simulink library "cvt_components_lib"  (R2025a)
settings: Solver=VariableStepAuto  StartTime=0.0  StopTime=10.0  RelTol=1e-3
undefined symbols (not defined in the file): HMPST
libraries: fl_lib x15, sdl_lib x5, nesl_utility x2, simulink_extras x1
Description:
  | Copyright 2023-2025 The MathWorks, Inc.
settings Model: Creator=smiller  LastModifiedBy=smiller
settings RTWCC: GPUComputeCapability=3.5

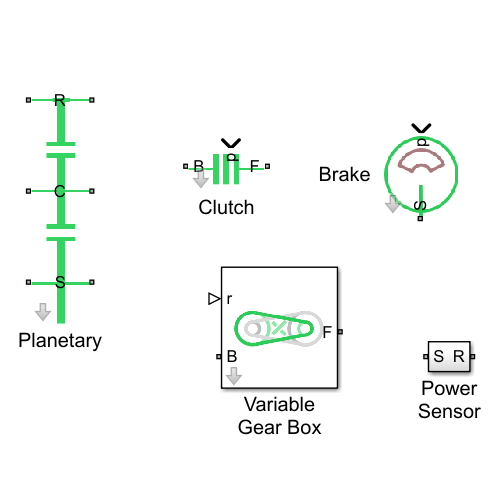
[thumbnail: Simulink's stored preview of the top-level diagram]
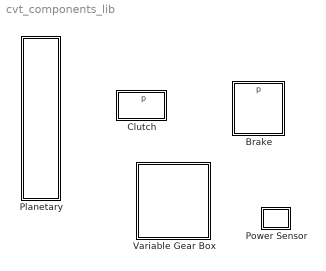
== system cvt_components_lib ==
  Brake : Subsystem  mask(Disk Brake){bore=HMPST.Brake.cylBore, brkwy_vel=HMPST.Brake.vBrk, mu_static=HMPST.Brake.muSta, mu_coulomb=HMPST.Brake.muKin, n_pads=HMPST.Brake.numPads, r_mean=HMPST.Brake.rPad, visc_coef=HMPST.Brake.dVisc, logic2pressure=HMPST.Brake.logic2Press, ts_filt=HMPST.Brake.tsFilt}
      mask prompts: bore "Cylinder bore"; brkwy_vel "Breakaway friction velocity"; mu_static "Static friction coefficient"; mu_coulomb "Coulomb friction coefficient"; n_pads "Number of brake pads"; r_mean "Mean pad radius"; visc_coef "Viscous friction coefficient"; logic2pressure "Logic to Pressure (Pa)"; ts_filt "Filter time constant (sec)"
      mask help: Models a disk brake. Brake actuation dynamics are modeled abstractly as a transfer function.
      mask TypeOptions bore: Brake/bore
      mask TypeOptions brkwy_vel: Brake/brkwy_vel
      mask TypeOptions mu_static: Brake/mu_static
      mask TypeOptions mu_coulomb: Brake/mu_coulomb
      mask TypeOptions n_pads: Brake/n_pads
      mask TypeOptions r_mean: Brake/r_mean
      mask TypeOptions visc_coef: Brake/visc_coef
      mask TypeOptions logic2pressure: Logic to Pressure/Gain
      mask Display: image('sm_wheel_loader_brake1D_IMAGE.png')
  Clutch : Subsystem  mask(Clutch){r_eff=200, nS=8, piston_area=0.0083, mu_static=0.6, mu_coulomb=0.4, w_tol=0.001, pressure_min=100, logic_to_pr_gain=10^6, ts_filt=0.05}
      mask prompts: r_eff "Effective torque radius (mm)"; nS "Number of friction surfaces"; piston_area "Engagement piston area (m^2)"; mu_static "Static friction coefficient (0-1)"; mu_coulomb "Kinetic friction coefficient (0-1)"; w_tol "Clutch velocity tolerance (rad/s)"; pressure_min "Engagement threshold pressure (Pa)"; logic_to_pr_gain "Logic to pressure gain (Pa)"; ts_filt "Filter time constant (sec)"
      mask help: Models a disk clutch. Clutch dynamics for engaging are modeled abstractly as a transfer function.
      settings: PortSchema="{\"entries\":[{\"content\":{\"sides\":[{\"content\":{\"connectorIds\":[\"LConn1\"]},\"type\":\"ConnectorPlacement.EquallySpacedRectSide\",\"uuid\":\"287225fd-8891-4f7c-8f3e-4b5002d781cc\"},{\"content\":{\"connectorIds\":[\"RConn1\"],\"side\":\"RIGHT\"},\"type\":\"ConnectorPlacement.EquallySpacedRectSide\",\"uuid\":\"52798522-6832-475b-a38f-3591fd9a4abf\"},{\"content\":{\"connectorIds\":[\"In1\"],\"side\":\"TOP\"},\"type\":\"ConnectorPlacement.EquallySpacedRectSide\",\"uuid\":\"1831134e-0a5d-4b10-be5a-e490a8ed770c\"}]},\"type\":\"ConnectorPlacement.EquallySpacedConnector\",\"uuid\":\"90a48bee-b3bb-49b8-9036-fc770fa0982b\"}],\"packageUris\":[\"http://schema.mathworks.com/mf0/Connector/R2020b\"],\"version\":\"1.0\"}"
      mask TypeOptions r_eff: Clutch/r_eff
      mask TypeOptions nS: Clutch/nS
      mask TypeOptions piston_area: Clutch/piston_area
      mask TypeOptions mu_static: Clutch/mu_static
      mask TypeOptions mu_coulomb: Clutch/mu_coulomb
      mask TypeOptions w_tol: Clutch/w_tol
      mask TypeOptions pressure_min: Clutch/pressure_min
      mask TypeOptions logic_to_pr_gain: Gain/Gain
      mask Display: image('sm_wheel_loader_clutch1D_IMAGE.png');
  Planetary : Subsystem  mask(Planetary Gear){rs_ratio=HMPST.GearTrain.PG1.Ring.TeethNum/HMPST.GearTrain.PG1.Sun.TeethNum, pg_efficiency=[.995, .995], ring_inertia=0.5, carr_inertia=0.5, sun_inertia=0.5, w_specify=on, w_priority=None, w=0}
      mask prompts: rs_ratio "Ring (R) to sun (S) teeth ratio (NR/NS)"; pg_efficiency "Efficiency [Sun-planet, ring-planet] (0-1)"; ring_inertia "Ring Inertia (kg*m^2)"; carr_inertia "Carrier Inertia (kg*m^2)"; sun_inertia "Sun Inertia (kg*m^2)"; w_specify "physmod:simscape:library:comments:mechanical:rotational:inertia:w"; w_priority "physmod:common:pi:sli:kernel:VariablePriority"; w "physmod:common:pi:sli:kernel:VariableValue"
      mask help: Models a planetary gear. Ports for the sun (S), carrier (C), and ring (R) are on both sides to simplify schematic assembly.
      mask TypeOptions rs_ratio: Planetary/rs_ratio
      mask TypeOptions pg_efficiency: Planetary/efficiency
      mask TypeOptions w_specify: Ring Inertia/w_specify
      mask TypeOptions w_priority: Ring Inertia/w_priority
      mask TypeOptions w: Ring Inertia/w
      mask DialogControl cont_ring_ic Prompt: Ring Inertia Initial Conditions
      mask DialogControl w_specify Prompt: Rotational velocity
      mask DialogControl w_priority Prompt: Priority
      mask DialogControl w Prompt: Value
      mask Display: image('sm_wheel_loader_planetary1D_IMAGE.png');
  Power Sensor : Subsystem
  Variable Gear Box : Subsystem  mask(Variable Ratio Gear Box){k=10000, d=100, dInput=0.01*2, dOutput=0.1*2}
      mask prompts: k "Compliance Stiffness (N*m/rad)"; d "Compliance Damping (N*m/(rad/s))"; dInput "Damping Coefficient Input (N*m/(rad/s))"; dOutput "Damping coefficient Output (N*m/(rad/s))"
      mask help: Models a variable ratio gear. The ratio can be negative, positive, or zero. Separate damping elements are connected to the input and output shafts to represent viscous friction. A small compliant element captures dynamics within the gear.
      mask TypeOptions dInput:
      | Input Shaft
      | Damper/D
      mask TypeOptions dOutput:
      | Output Shaft
      | Damper/D
      mask Display: image('ssc_variable_gear_box_IMAGE.png')

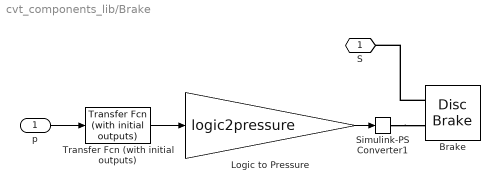
== system cvt_components_lib/Brake ==
  p : Inport
  Brake : sdl_lib/Brakes & Detents/Rotational/Disc Brake  r_mean=r_mean mm  bore=bore mm  n_pads=n_pads  thermal_port=simscape.enum.thermaleffects.omit  mu_static=mu_static  mu_coulomb=mu_coulomb  temperature_TLU=[280, 300, 320] K  mu_static_TLU=[.9, .8, .7]  mu_coulomb_TLU=[.8, .7, .6]  brkwy_vel=brkwy_vel rad/s  visc_coef=visc_coef N*m*s/rad  thermal_mass=50 kJ/K  temperature_specify=off  temperature_priority=High  temperature=300 K  temperature_nominal_specify=off  temperature_nominal_value=1  temperature_nominal_unit=K
  Logic to Pressure : Gain  Gain=logic2pressure
  Simulink-PS Converter1 : nesl_utility/Simulink-PS Converter  PhysicalDomain=network_engine_domain  SubClassName=ps_input  LeftPortType=input  RightPortType=output  PseudoPeriodic=off  Frequencies=[]  NoiseDistribution=none  NoiseParameters=[]  Unit=1  AffineConversion=off  FilteringAndDerivatives=provide  SimscapeFilterOrder=1  InputFilterTimeConstant=0.001  UdotUserProvided=0
  Transfer Fcn (with initial outputs) : simulink_extras/Additional Linear/Transfer Fcn (with initial outputs)  N=1  D=[ts_filt 1]  Y0=0  U0=0
  S : PMIOPort  Side=Right
  wires:
  Transfer Fcn (with initial outputs)/1 -> Logic to Pressure/1
  Logic to Pressure/1 -> Simulink-PS Converter1/1
  p/1 -> Transfer Fcn (with initial outputs)/1
  connections:
  Brake/LConn2 -- S/RConn1
  Simulink-PS Converter1/RConn1 -- Brake/LConn1

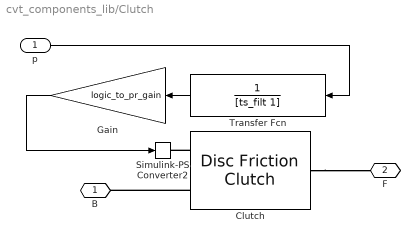
== system cvt_components_lib/Clutch ==
  p : Inport
  Clutch : sdl_lib/Clutches/Disc Friction Clutch  geometry_model=1  r_eff=r_eff mm  d_o=150 mm  d_i=100 mm  nS=nS  piston_area=piston_area m^2  unidirectional=0  friction_model=1  mu_w_vector=[ 0 0.1 0.2 0.3 0.4 0.5 1 2 5 10 100 1000 ] rad/s  temperature_TLU=[280.0, 300.0, 320.0] K  mu_static=mu_static  mu_static_vector=[0.4, 0.38, 0.36]  mu_coulomb=mu_coulomb  mu_coulomb_vector=[ 0.29 0.28 0.26 0.22 0.21 0.2 0.2 0.19 0.19 0.19 0.19 0.19 ]  mu_coulomb_temp_vector=[0.3, 0.28, 0.25]  mu_coulomb_matrix=[0.34, 0.32, 0.3; 0.3, 0.28, 0.25; 0.25, 0.2, 0.15]  mu_interp_method=1  mu_extrap_method=1  d_f=1  w_tol=w_tol rad/s  pressure_min=pressure_min Pa  mu_visc=0 N*m/(rad/s)  initial_state_locked=0  thermal_mass=25 kJ/K  T_init=300 K
      settings: InternalSimscapePortConfiguration="{\"Bottom\":[],\"Left\":[{\"id\":\"P\",\"label\":\"P\",\"type\":\"input\"},{\"id\":\"B\",\"label\":\"B\",\"type\":\"foundation.mechanical.rotational.rotational\"}],\"Right\":[{\"id\":\"F\",\"label\":\"F\",\"type\":\"foundation.mechanical.rotational.rotational\"}],\"Top\":[]}"
  Gain : Gain  Gain=logic_to_pr_gain
  Simulink-PS Converter2 : nesl_utility/Simulink-PS Converter  PhysicalDomain=network_engine_domain  SubClassName=ps_input  LeftPortType=input  RightPortType=output  PseudoPeriodic=off  Frequencies=[]  NoiseDistribution=none  NoiseParameters=[]  Unit=1  AffineConversion=off  FilteringAndDerivatives=provide  SimscapeFilterOrder=1  InputFilterTimeConstant=0.001  UdotUserProvided=0
  Transfer Fcn : TransferFcn  Numerator=1  Denominator=[ts_filt 1]
  B : PMIOPort  Side=Left
  F : PMIOPort  Port=2  Side=Right
  wires:
  Gain/1 -> Simulink-PS Converter2/1
  Transfer Fcn/1 -> Gain/1
  p/1 -> Transfer Fcn/1
  connections:
  Clutch/LConn1 -- Simulink-PS Converter2/RConn1
  Clutch/RConn1 -- F/RConn1
  Clutch/LConn2 -- B/RConn1

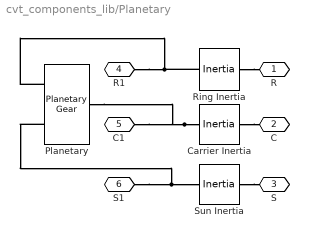
== system cvt_components_lib/Planetary ==
  Carrier Inertia : fl_lib/Mechanical/Rotational Elements/Inertia  inertia=carr_inertia kg*m^2  num_ports=foundation.enum.numPorts2.two  w_specify=on  w_priority=None  w=0 rad/s  w_nominal_specify=off  w_nominal_value=1  w_nominal_unit=rad/s  t_specify=off  t_priority=None  t=0 N*m  t_nominal_specify=off  t_nominal_value=1  t_nominal_unit=N*m
      settings: InternalSimscapePortConfiguration="{\"Bottom\":[],\"Left\":[{\"id\":\"I\",\"label\":\"\",\"type\":\"foundation.mechanical.rotational.rotational\"}],\"Right\":[{\"id\":\"J\",\"label\":\"\",\"type\":\"foundation.mechanical.rotational.rotational\"}],\"Top\":[]}"
  Planetary : sdl_lib/Gears/Planetary Gear  rs_ratio=rs_ratio  friction_model=sdl.enum.gear_friction.constant  efficiency=pg_efficiency  temperature_TLU=[280, 300, 320] K  efficiency_sp_TLU=[.95, .9, .85]  efficiency_rp_TLU=[.95, .9, .85]  pwr_thr=[.001, .001] W  mu_visc=[0, 0] N*m*s/rad  model_inertia=simscape.enum.onoff.off  sun_inertia=1e-10 kg*m^2  ring_inertia=1e-10 kg*m^2  carrier_inertia=1e-10 kg*m^2  carrier_radius=0.01 m  planet_inertia=0.001 kg*m^2  planet_mass=1e-10 kg  thermal_mass=50 J/K  T_init=300 K
  Ring Inertia : fl_lib/Mechanical/Rotational Elements/Inertia  inertia=ring_inertia kg*m^2  num_ports=foundation.enum.numPorts2.two  w_specify=on  w_priority=None  w=w rad/s  w_nominal_specify=off  w_nominal_value=1  w_nominal_unit=rad/s  t_specify=off  t_priority=None  t=0 N*m  t_nominal_specify=off  t_nominal_value=1  t_nominal_unit=N*m
      settings: InternalSimscapePortConfiguration="{\"Bottom\":[],\"Left\":[{\"id\":\"I\",\"label\":\"\",\"type\":\"foundation.mechanical.rotational.rotational\"}],\"Right\":[{\"id\":\"J\",\"label\":\"\",\"type\":\"foundation.mechanical.rotational.rotational\"}],\"Top\":[]}"
  Sun Inertia : fl_lib/Mechanical/Rotational Elements/Inertia  inertia=sun_inertia kg*m^2  num_ports=foundation.enum.numPorts2.two  w_specify=on  w_priority=None  w=0 rad/s  w_nominal_specify=off  w_nominal_value=1  w_nominal_unit=rad/s  t_specify=off  t_priority=None  t=0 N*m  t_nominal_specify=off  t_nominal_value=1  t_nominal_unit=N*m
      settings: InternalSimscapePortConfiguration="{\"Bottom\":[],\"Left\":[{\"id\":\"I\",\"label\":\"\",\"type\":\"foundation.mechanical.rotational.rotational\"}],\"Right\":[{\"id\":\"J\",\"label\":\"\",\"type\":\"foundation.mechanical.rotational.rotational\"}],\"Top\":[]}"
  "R    " : PMIOPort  Side=Right
  "C    " : PMIOPort  Port=2  Side=Right
  "S    " : PMIOPort  Port=3  Side=Right
  R1 : PMIOPort  Port=4  Side=Left
  C1 : PMIOPort  Port=5  Side=Left
  S1 : PMIOPort  Port=6  Side=Left
  connections:
  Planetary/RConn2 -- S1/RConn1 -- Sun Inertia/RConn1
  Carrier Inertia/RConn1 -- Planetary/LConn1 -- C1/RConn1
  Planetary/RConn1 -- Ring Inertia/RConn1 -- R1/RConn1
  Carrier Inertia/LConn1 -- "C    "/RConn1
  Ring Inertia/LConn1 -- "R    "/RConn1
  Sun Inertia/LConn1 -- "S    "/RConn1

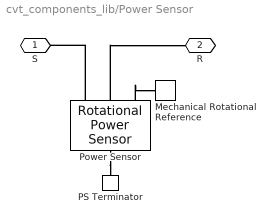
== system cvt_components_lib/Power Sensor ==
  Mechanical Rotational Reference : fl_lib/Mechanical/Rotational Elements/Mechanical Rotational Reference
  PS Terminator : fl_lib/Physical Signals/Sinks/PS Terminator
  Power Sensor : sdl_lib/Sensors/Rotational Power Sensor  measurement_type=sdl.enum.rotationalPowerSensorType.instantaneous  averaging_period=1 s  max_frequency=1000 Hz  max_speed=1000 rpm
      settings: InternalSimscapePortConfiguration="{\"Bottom\":[],\"Left\":[{\"id\":\"S\",\"label\":\"S\",\"type\":\"foundation.mechanical.rotational.rotational\"},{\"id\":\"R\",\"label\":\"R\",\"type\":\"foundation.mechanical.rotational.rotational\"},{\"id\":\"C\",\"label\":\"C\",\"type\":\"foundation.mechanical.rotational.rotational\"}],\"Right\":[{\"id\":\"P\",\"label\":\"P\",\"type\":\"output\"}],\"Top\":[]}"
  S : PMIOPort  Side=Left
  R : PMIOPort  Port=2  Side=Right
  connections:
  Power Sensor/RConn1 -- PS Terminator/LConn1
  Power Sensor/LConn3 -- Mechanical Rotational Reference/LConn1
  Power Sensor/LConn2 -- R/RConn1
  Power Sensor/LConn1 -- S/RConn1

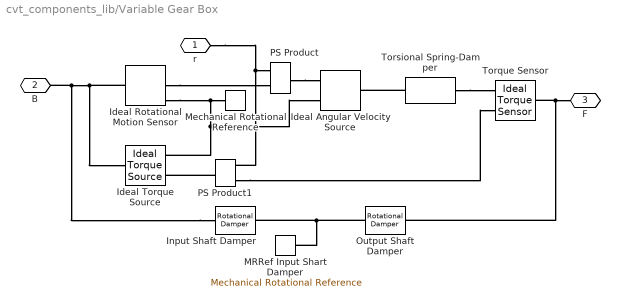
== system cvt_components_lib/Variable Gear Box ==
  Ideal Angular Velocity Source : fl_lib/Mechanical/Mechanical Sources/Ideal Angular Velocity Source
  Ideal Rotational Motion Sensor : fl_lib/Mechanical/Mechanical Sensors/Ideal Rotational Motion Sensor  reference=foundation.enum.MeasurementReference.difference  acceleration_port=false  velocity_port=true  position_port=true  wrap_angle=false  offset=0 rad
  Ideal Torque Source : fl_lib/Mechanical/Mechanical Sources/Ideal Torque Source
  Input Shaft Damper : fl_lib/Mechanical/Rotational Elements/Rotational Damper  D=dInput N*m/(rad/s)  w_specify=off  w_priority=High  w=0 rad/s  w_nominal_specify=off  w_nominal_value=1  w_nominal_unit=rad/s  t_specify=off  t_priority=High  t=0 N*m  t_nominal_specify=off  t_nominal_value=1  t_nominal_unit=N*m
  MRRef Input Shart Damper : fl_lib/Mechanical/Rotational Elements/Mechanical Rotational Reference
  Mechanical Rotational Reference : fl_lib/Mechanical/Rotational Elements/Mechanical Rotational Reference
  Output Shaft Damper : fl_lib/Mechanical/Rotational Elements/Rotational Damper  D=dOutput N*m/(rad/s)  w_specify=off  w_priority=High  w=0 rad/s  w_nominal_specify=off  w_nominal_value=1  w_nominal_unit=rad/s  t_specify=off  t_priority=High  t=0 N*m  t_nominal_specify=off  t_nominal_value=1  t_nominal_unit=N*m
  PS Product : fl_lib/Physical Signals/Functions/PS Product
  PS Product1 : fl_lib/Physical Signals/Functions/PS Product
  Torque Sensor : fl_lib/Mechanical/Mechanical Sensors/Ideal Torque Sensor
  Torsional Spring-Damper : sdl_lib/Couplings & Drives/Torsional Spring-Damper  k=k N*m/rad  mu_visc=d N*m*s/rad  trq_coulomb=0 N*m  static_kinetic_ratio=1.1  w_tol=0.001 rad/s  model_hardstop=sdl.enum.hardStopOffOn.off  upper_bound=10 deg  lower_bound=-10 deg  hardstop_model=simscape.enum.hardstop.smooth  k_endstop=1e6 N*m/rad  D_endstop=10 N*m*s/rad  transition=0.001 rad  coeff_rest=0.7  w_tol_hardstop=0.1 rad/s  trq_tol=0.001 N*m  x0=0 deg
      settings: InternalSimscapePortConfiguration="{\"Bottom\":[],\"Left\":[{\"id\":\"R\",\"label\":\"R\",\"type\":\"foundation.mechanical.rotational.rotational\"}],\"Right\":[{\"id\":\"C\",\"label\":\"C\",\"type\":\"foundation.mechanical.rotational.rotational\"}],\"Top\":[]}"
  r : PMIOPort  Side=Left
  B : PMIOPort  Port=2  Side=Left
  F : PMIOPort  Port=3  Side=Right
  connections:
  Ideal Rotational Motion Sensor/RConn1 -- Mechanical Rotational Reference/LConn1 -- Ideal Angular Velocity Source/RConn2 -- Ideal Torque Source/RConn2
  Ideal Rotational Motion Sensor/RConn2 -- PS Product/LConn2
  PS Product/RConn1 -- Ideal Angular Velocity Source/RConn1
  PS Product1/LConn2 -- Torque Sensor/RConn2
  Torsional Spring-Damper/RConn1 -- Torque Sensor/RConn1
  Torsional Spring-Damper/LConn1 -- Ideal Angular Velocity Source/LConn1
  PS Product1/RConn1 -- Ideal Torque Source/RConn1
  Output Shaft Damper/RConn1 -- Input Shaft Damper/RConn1 -- MRRef Input Shart Damper/LConn1
  Output Shaft Damper/LConn1 -- F/RConn1 -- Torque Sensor/LConn1
  Input Shaft Damper/LConn1 -- B/RConn1 -- Ideal Rotational Motion Sensor/LConn1 -- Ideal Torque Source/LConn1
  PS Product1/LConn1 -- r/RConn1 -- PS Product/LConn1
